simulink model "HeartExe_second"  (R2023b)
settings: Solver=ode1  StartTime=0.0  StopTime=30.0  FixedStep=0.5e-3  RelTol=1e-3
model workspace: external: MAT-File N3Data_second.mat (data not in the file)
libraries: Libs_second x151
(part 1 of 3)
settings Model: SimulationMode=accelerator  Creator=wai484  LastModifiedBy=wai484
settings SolverCC: AlgebraicLoopSolver=TrustRegion
settings DataIOCC: SaveOutput=off  SignalLogging=off  DSMLogging=off  SaveTime=off  ReturnWorkspaceOutputs=off
settings DebuggingCC: UnconnectedInputMsg=warning  UnconnectedOutputMsg=warning  UnconnectedLineMsg=warning  ArithmeticOperatorsInVariantConditions=warning
settings ModelReferenceCC: EnableRefExpFcnMdlSchedulingChecks=on
settings SFSimCC: SimUseLocalCustomCode=off  CustomCodeUndefinedFunction=UseInterfaceOnly
settings RTWCC: RTWUseLocalCustomCode=off  BuildConfiguration=Faster Runs
settings CodeAppCC: StateflowObjectComments=on

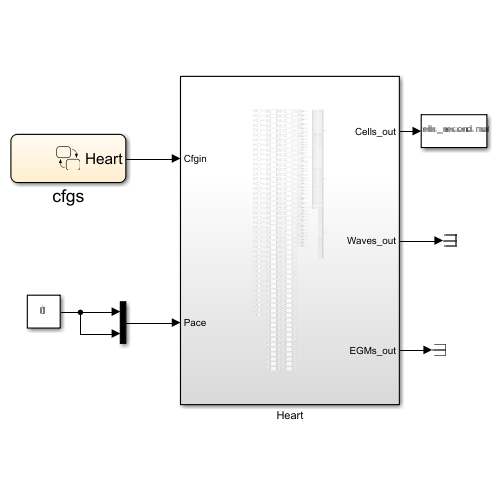
[thumbnail: Simulink's stored preview of the top-level diagram]
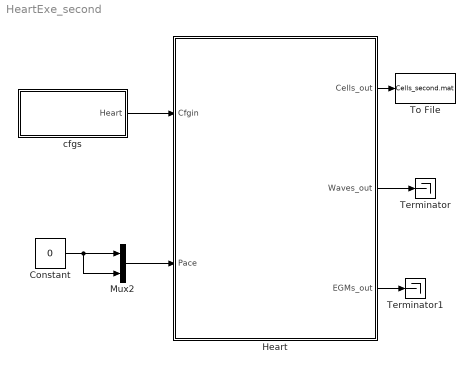
== system HeartExe_second ==
  Constant : Constant  Value=0
  Heart : Subsystem
  Mux2 : Mux  Inputs=2
  Terminator : Terminator
  Terminator1 : Terminator
  To File : ToFile  Filename=Cells_second.mat  MatrixName=cells
  cfgs : Stateflow chart  TreatAsAtomicUnit=on
  wires:
  cfgs/1(Heart) -> Heart/1(Cfgin)
  Mux2/1 -> Heart/2(Pace)
  Constant/1 -> Mux2/2, Mux2/1
  Heart/2(Waves_out) -> Terminator/1
  Heart/3(EGMs_out) -> Terminator1/1
  Heart/1(Cells_out) -> To File/1
